simulink library "Lib_Piccolo"  (R2018b)
settings: Solver=VariableStepAuto  StartTime=0.0  StopTime=10.0  RelTol=1e-3
values from neighbouring files (symbols this model uses):
  AccelErrInt2Brakes = 0.15    [SimulationControlConfig16P.m]    (also in SimulationControlConfig16P_LEGACY.m; SimulationControlConfigTAILLESS.m = 0.2; SimulationControlConfigUTAIL.m = 0.2)
  AileronMax = 25    [SimulationControlConfig16P.m]    (also in SimulationControlConfig16P_LEGACY.m; SimulationControlConfigTAILLESS.m; SimulationControlConfigUTAIL.m)
  AileronPower = 0.00268    [SimulationControlConfig16P.m]    (also in SimulationControlConfig16P_LEGACY.m; SimulationControlConfigTAILLESS.m; SimulationControlConfigUTAIL.m)
  AileronSurfaceMax = 45    [SimulationControlConfig16P.m]    (also in SimulationControlConfig16P_LEGACY.m)
  AileronTrim = 0    [SimulationControlConfig16P.m]    (also in SimulationControlConfig16P_LEGACY.m; SimulationControlConfigTAILLESS.m; SimulationControlConfigUTAIL.m)
  Alt = 1000 + TerrainHeight    [SimulationStateConfig.m]
  AltCruise_m = testPlans(testIndx).terrainElevation * 0.3048 + 200    [SimulationControlConfig16P.m]    (also in SimulationControlConfigTAILLESS.m = 1083; SimulationControlConfigUTAIL.m = testPlans(testIndx).terrainElevation * 0.3048 + 152)
  AltitudeRate2PitchCmdIntegratorInit = 0.1    [SimulationControlPre.m]
  AltMax = 10000    [SimulationControlConfig16P.m]    (also in SimulationControlConfig16P_LEGACY.m; SimulationControlConfigTAILLESS.m; SimulationControlConfigUTAIL.m)
  AltMaxAccel = 1.25    [SimulationControlConfig16P.m]    (also in SimulationControlConfig16P_LEGACY.m = 0.9; SimulationControlConfigTAILLESS.m = 1.7; SimulationControlConfigUTAIL.m = 2)
  AltMin = 0    [SimulationControlConfig16P.m]    (also in SimulationControlConfig16P_LEGACY.m; SimulationControlConfigTAILLESS.m; SimulationControlConfigUTAIL.m)
  AltRateCmd2Pitch = 0.50    (= 0.5)    [SimulationControlConfig16P.m]    (also in SimulationControlConfig16P_LEGACY.m = 0.6; SimulationControlConfigTAILLESS.m = 0.2; SimulationControlConfigUTAIL.m = 0.3)
  AltRateError2Pitch = 0.40    (= 0.4)    [SimulationControlConfig16P.m]    (also in SimulationControlConfig16P_LEGACY.m; SimulationControlConfigTAILLESS.m = 0.55; SimulationControlConfigUTAIL.m = 0.55)
  AltRateErrorInt2Pitch = 0.50    (= 0.5)    [SimulationControlConfig16P.m]    (also in SimulationControlConfig16P_LEGACY.m = 0.45; SimulationControlConfigTAILLESS.m; SimulationControlConfigUTAIL.m = 0.75)
  AltRateLpfCutOff = 3    [SimulationControlConfig16P.m]    (also in SimulationControlConfig16P_LEGACY.m; SimulationControlConfigTAILLESS.m = 2; SimulationControlConfigUTAIL.m = 2)
  AutoNosegear2Rudder = 26    [SimulationControlConfig16P.m]    (also in SimulationControlConfig16P_LEGACY.m; SimulationControlConfigTAILLESS.m = 25.2; SimulationControlConfigUTAIL.m = 14)
  b = 5.54    [SimulationControlConfig16P.m]    (also in SimulationControlConfig16P_LEGACY.m; SimulationControlConfigTAILLESS.m = 2.37; SimulationControlConfigUTAIL.m = 2.37)
  Bank2AileronIntegratorInit = 0    [SimulationControlPre.m]
  BankMax_User = BankMax_User/180*pi    (= 0.523598775598)    [SimulationControlConfig16P.m]    (also in SimulationControlConfig16P_LEGACY.m; SimulationControlConfigTAILLESS.m = 0.610865238198; SimulationControlConfigUTAIL.m = 0.628318530718)
  baseLegFlaps = 20    [SimulationControlConfig16P.m]    (also in SimulationControlConfig16P_LEGACY.m = 0; SimulationControlConfigTAILLESS.m = 15; SimulationControlConfigUTAIL.m = 10)
  C = GeneticOpt.C    [SimulationCostFunction.m]
  c = Sw/b    (= 0.841696750903)    [SimulationControlConfig16P.m]    (also in SimulationControlConfig16P_LEGACY.m; SimulationControlConfigTAILLESS.m = 0.354008438819; SimulationControlConfigUTAIL.m = 0.354008438819)
  cell2WheelFactorMG = 5.98    [SimulationSensorConfig16P_LEGACY.m]
  cell2WheelFactorNG = 1    [SimulationSensorConfig16P_LEGACY.m]
  cellSatMaxMG = 15000    [SimulationSensorConfig16P.m]    (also in SimulationSensorConfig16P_LEGACY.m; SimulationSensorConfigTAILLESS7P.m; SimulationSensorConfigUTAIL7P.m)
  cellSatMaxNG = 1000    [SimulationSensorConfig16P.m]    (also in SimulationSensorConfig16P_LEGACY.m; SimulationSensorConfigTAILLESS7P.m; SimulationSensorConfigUTAIL7P.m)
  cellSatMinMG = -15000    [SimulationSensorConfig16P.m]    (also in SimulationSensorConfig16P_LEGACY.m; SimulationSensorConfigTAILLESS7P.m; SimulationSensorConfigUTAIL7P.m)
  cellSatMinNG = -1000    [SimulationSensorConfig16P.m]    (also in SimulationSensorConfig16P_LEGACY.m; SimulationSensorConfigTAILLESS7P.m; SimulationSensorConfigUTAIL7P.m)
  CL_Limit = CL_Max    (= 0.54)    [SimulationControlConfig16P.m]    (also in SimulationControlConfig16P_LEGACY.m; SimulationControlConfigTAILLESS.m; SimulationControlConfigUTAIL.m = 0.53)
  CL_Max = 0.54    [SimulationControlConfig16P.m]    (also in SimulationControlConfig16P_LEGACY.m; SimulationControlConfigTAILLESS.m; SimulationControlConfigUTAIL.m = 0.53)
  CL_Max_Nom = 0.465    [SimulationControlConfig16P.m]    (also in SimulationControlConfig16P_LEGACY.m; SimulationControlConfigTAILLESS.m = 0.39; SimulationControlConfigUTAIL.m)
  CL_Min = 0    [SimulationControlConfig16P.m]    (also in SimulationControlConfig16P_LEGACY.m; SimulationControlConfigTAILLESS.m; SimulationControlConfigUTAIL.m)
  ClimbMaxFraction = 0.35    [SimulationControlConfig16P.m]    (also in SimulationControlConfig16P_LEGACY.m = 0.24; SimulationControlConfigTAILLESS.m = 0.19; SimulationControlConfigUTAIL.m = 0.21)
  ClimboutMaxBank = 7.0    (= 7)    [SimulationControlConfig16P.m]    (also in SimulationControlConfig16P_LEGACY.m; SimulationControlConfigTAILLESS.m = 5; SimulationControlConfigUTAIL.m)
  ClimboutTimer = 7.0    (= 7)    [SimulationControlConfig16P.m]    (also in SimulationControlConfig16P_LEGACY.m; SimulationControlConfigTAILLESS.m; SimulationControlConfigUTAIL.m)
  dCl_per_dFlap = 0.005581818    [SimulationControlConfig16P.m]    (also in SimulationControlConfig16P_LEGACY.m = 0; SimulationControlConfigTAILLESS.m = 0; SimulationControlConfigUTAIL.m = 0)
  DecelerationCmd = 3.1    [SimulationControlConfig16P.m]    (also in SimulationControlConfig16P_LEGACY.m; SimulationControlConfigTAILLESS.m = 0.1; SimulationControlConfigUTAIL.m = 0.1)
  DeRotateLogicEndTimer = abs((NoseDownLimit_Deg-1)/DeRotateRamp_Dps)    [SimulationControlConfig16P.m]    (also in SimulationControlConfig16P_LEGACY.m; SimulationControlConfigTAILLESS.m; SimulationControlConfigUTAIL.m)
  DeRotateLogicHoldNoseUpTimer = 0.1    [SimulationControlConfig16P.m]    (also in SimulationControlConfig16P_LEGACY.m; SimulationControlConfigTAILLESS.m; SimulationControlConfigUTAIL.m)
  DeRotateLogicTimerTimeout = 2    [SimulationControlConfig16P.m]    (also in SimulationControlConfig16P_LEGACY.m; SimulationControlConfigTAILLESS.m; SimulationControlConfigUTAIL.m)
  DeRotateLowerCmdSaturation = 0    [SimulationControlConfig16P.m]    (also in SimulationControlConfig16P_LEGACY.m; SimulationControlConfigTAILLESS.m; SimulationControlConfigUTAIL.m)
  DeRotateRamp_Dps = 3    [SimulationControlConfig16P.m]    (also in SimulationControlConfig16P_LEGACY.m; SimulationControlConfigTAILLESS.m = 8; SimulationControlConfigUTAIL.m = 8)
  DeRotateUpperCmdSaturation = 7    [SimulationControlConfig16P.m]    (also in SimulationControlConfig16P_LEGACY.m; SimulationControlConfigTAILLESS.m; SimulationControlConfigUTAIL.m)
  DescentMaxFraction = 0.22    [SimulationControlConfig16P.m]    (also in SimulationControlConfig16P_LEGACY.m = 0.2; SimulationControlConfigTAILLESS.m = 0.17; SimulationControlConfigUTAIL.m = 0.17)
  DesktopSimTerrainOffset_m = 0.406    [SimulationAircraftConfig.m]
  downwindFlaps = 0    [SimulationControlConfig16P.m]    (also in SimulationControlConfig16P_LEGACY.m; SimulationControlConfigTAILLESS.m; SimulationControlConfigUTAIL.m)
  DP_init = 0.5*1.225*V_init^2    [SimulationControlConfig16P.m]    (also in SimulationControlConfig16P_LEGACY.m; SimulationControlConfigTAILLESS.m; SimulationControlConfigUTAIL.m)
  dscNoiseMG = 1    [SimulationSensorConfig16P_LEGACY.m]
  dscNoiseNG = 0.25    [SimulationSensorConfig16P_LEGACY.m]
  DSCnumBits = 24    [SimulationSensorConfig16P.m]    (also in SimulationSensorConfig16P_LEGACY.m; SimulationSensorConfigTAILLESS7P.m; SimulationSensorConfigUTAIL7P.m)
  DSCRangeMaxMG = 15000    [SimulationSensorConfig16P.m]    (also in SimulationSensorConfig16P_LEGACY.m; SimulationSensorConfigTAILLESS7P.m; SimulationSensorConfigUTAIL7P.m)
  DSCRangeMaxNG = 1000    [SimulationSensorConfig16P.m]    (also in SimulationSensorConfig16P_LEGACY.m; SimulationSensorConfigTAILLESS7P.m; SimulationSensorConfigUTAIL7P.m)
  DSCRangeMinMG = -15000    [SimulationSensorConfig16P.m]    (also in SimulationSensorConfig16P_LEGACY.m; SimulationSensorConfigTAILLESS7P.m; SimulationSensorConfigUTAIL7P.m)
  DSCRangeMinNG = -1000    [SimulationSensorConfig16P.m]    (also in SimulationSensorConfig16P_LEGACY.m; SimulationSensorConfigTAILLESS7P.m; SimulationSensorConfigUTAIL7P.m)
  dt = DLLSim.dt    [SimulationTimeStep.m]    (also in SimulationTrim.m = 0.02)
  EarlyTouchdownThreshold = 3.0    (= 3)    [SimulationControlConfig16P.m]    (also in SimulationControlConfig16P_LEGACY.m; SimulationControlConfigTAILLESS.m = 2.2; SimulationControlConfigUTAIL.m = 2.5)
  ElevatorDeflectionRate = 15    [SimulationControlConfig16P.m]    (also in SimulationControlConfig16P_LEGACY.m = 12; SimulationControlConfigTAILLESS.m = 10; SimulationControlConfigUTAIL.m = 12)
  ElevatorMax = 25    [SimulationControlConfig16P.m]    (also in SimulationControlConfig16P_LEGACY.m; SimulationControlConfigTAILLESS.m; SimulationControlConfigUTAIL.m)
  ElevatorPower = -0.002209    [SimulationControlConfig16P.m]    (also in SimulationControlConfig16P_LEGACY.m; SimulationControlConfigTAILLESS.m = -0.002956; SimulationControlConfigUTAIL.m = -0.00205983)
  ElevatorTrim = -3.5    [SimulationControlConfig16P.m]    (also in SimulationControlConfig16P_LEGACY.m; SimulationControlConfigTAILLESS.m = -6; SimulationControlConfigUTAIL.m = -8)
  elevonBias = 0    [SimulationControlConfig16P.m]    (also in SimulationControlConfig16P_LEGACY.m; SimulationControlConfigTAILLESS.m; SimulationControlConfigUTAIL.m)
  Enable_TAS_Protection = 0    [SimulationControlConfig16P.m]    (also in SimulationControlConfig16P_LEGACY.m; SimulationControlConfigTAILLESS.m; SimulationControlConfigUTAIL.m)
  EnableCrossTrackAbort = 1    [SimulationControlConfig16P.m]    (also in SimulationControlConfigTAILLESS.m; SimulationControlConfigUTAIL.m)
  EnergyBandwidth = 0.02    [SimulationControlConfig16P.m]    (also in SimulationControlConfig16P_LEGACY.m; SimulationControlConfigTAILLESS.m = 0.06; SimulationControlConfigUTAIL.m = 0.06)
  EngineLhFuelCut = 0    [SimulationAircraftConfig.m]
  EngineRhFuelCut = 0    [SimulationAircraftConfig.m]
  FastThrottleRate = 0.075    [SimulationControlConfig16P.m]    (also in SimulationControlConfig16P_LEGACY.m = 0.05; SimulationControlConfigTAILLESS.m = 0.1; SimulationControlConfigUTAIL.m = 0.1)
  FilterWarmUpTime = 2    [SimulationSensorConfig16P.m]    (also in SimulationSensorConfig16P_LEGACY.m; SimulationSensorConfigTAILLESS7P.m; SimulationSensorConfigUTAIL7P.m)
  finalApproachFlaps = 20    [SimulationControlConfig16P.m]    (also in SimulationControlConfig16P_LEGACY.m = 0; SimulationControlConfigTAILLESS.m = 22; SimulationControlConfigUTAIL.m = 10)
  FinalDescentSlope_Deg = testPlans(testIndx).descentSlope    [SimulationControlConfig16P.m]    (also in SimulationControlConfig16P_LEGACY.m; SimulationControlConfigTAILLESS.m; SimulationControlConfigUTAIL.m)
  flapMax = 0    [SimulationControlConfig16P.m]    (also in SimulationControlConfig16P_LEGACY.m; SimulationControlConfigTAILLESS.m; SimulationControlConfigUTAIL.m)
  flapRate = 7.5    [SimulationControlConfig16P.m]    (also in SimulationControlConfig16P_LEGACY.m; SimulationControlConfigTAILLESS.m = 6.6; SimulationControlConfigUTAIL.m)
  FlareHeight = 5    [SimulationControlConfig16P.m]    (also in SimulationControlConfig16P_LEGACY.m = 4.8; SimulationControlConfigTAILLESS.m = 2.5; SimulationControlConfigUTAIL.m = 2)
  FlareVerticalRate_mps = -0.4    [SimulationControlConfig16P.m]    (also in SimulationControlConfig16P_LEGACY.m = -0.5; SimulationControlConfigTAILLESS.m = -0.15; SimulationControlConfigUTAIL.m = -0.15)
  Fp_Aileron = 0.55*2*pi*RollRateLpfCutoff*dt    [SimulationControlConfig16P.m]    (also in SimulationControlConfig16P_LEGACY.m; SimulationControlConfigTAILLESS.m; SimulationControlConfigUTAIL.m)
  Fp_Alt = 0.55*AltBandwidth    (= 0.099)    [SimulationControlConfig16P.m]    (also in SimulationControlConfig16P_LEGACY.m; SimulationControlConfigTAILLESS.m = 0.587477826221; SimulationControlConfigUTAIL.m = 0.69115038379)
  Fp_AltRate = 0.55*2*pi*AltRateLpfCutOff*dt    [SimulationControlConfig16P.m]    (also in SimulationControlConfig16P_LEGACY.m; SimulationControlConfigTAILLESS.m; SimulationControlConfigUTAIL.m)
  Fp_Elevator = 0.55*2*pi*PitchRateLpfCutoff*dt    [SimulationControlConfig16P.m]    (also in SimulationControlConfig16P_LEGACY.m; SimulationControlConfigTAILLESS.m; SimulationControlConfigUTAIL.m)
  Fp_Energy = 0.55*2*pi*EnergyBandwidth    (= 0.069115038379)    [SimulationControlConfig16P.m]    (also in SimulationControlConfig16P_LEGACY.m; SimulationControlConfigTAILLESS.m = 0.207345115137; SimulationControlConfigUTAIL.m = 0.207345115137)
  Fp_Energy2 = 0.55*2*pi*EnergyBandwidth*dt    [SimulationControlConfig16P.m]    (also in SimulationControlConfig16P_LEGACY.m; SimulationControlConfigTAILLESS.m; SimulationControlConfigUTAIL.m)
  Fp_Pitch = 0.55*2*pi*PitchBandwidth    (= 2.76460153516)    [SimulationControlConfig16P.m]    (also in SimulationControlConfig16P_LEGACY.m = 3.11017672705; SimulationControlConfigTAILLESS.m = 3.80132711084; SimulationControlConfigUTAIL.m = 2.41902634326)
  Fp_Pitch_2 = 0.55*2*pi*PitchBandwidth*dt    [SimulationControlConfig16P.m]    (also in SimulationControlConfig16P_LEGACY.m; SimulationControlConfigTAILLESS.m; SimulationControlConfigUTAIL.m)
  Fp_Roll = RollBandwidth^2    (= 1)    [SimulationControlConfig16P.m]    (also in SimulationControlConfig16P_LEGACY.m = 1.44; SimulationControlConfigTAILLESS.m; SimulationControlConfigUTAIL.m)
  Fp_Rudder = 0.55*2*pi*YawRateLpfCutoff*dt    [SimulationControlConfig16P.m]    (also in SimulationControlConfig16P_LEGACY.m; SimulationControlConfigTAILLESS.m; SimulationControlConfigUTAIL.m)
  Fp_TAS = 0.55*2*pi*TASBandwidth    (= 0.103672557568)    [SimulationControlConfig16P.m]    (also in SimulationControlConfig16P_LEGACY.m; SimulationControlConfigTAILLESS.m = 0.172787595947; SimulationControlConfigUTAIL.m = 0.172787595947)
  Fp_TAS_Filter = 2*pi*TasLpfCutoff*dt    [SimulationControlConfig16P.m]    (also in SimulationControlConfig16P_LEGACY.m; SimulationControlConfigTAILLESS.m; SimulationControlConfigUTAIL.m)
  Fp_Turn = 0.55*2*pi*TurnErrLPFcutoff    (= 0.0345575191895)    [SimulationControlConfig16P.m]    (also in SimulationControlConfig16P_LEGACY.m; SimulationControlConfigTAILLESS.m = 0.172787595947; SimulationControlConfigUTAIL.m = 0.172787595947)
  Fp_TurnDerr = 0.55*2*pi*TurnDerivativeLPFcutoff    (= 0.0345575191895)    [SimulationControlConfig16P.m]    (also in SimulationControlConfig16P_LEGACY.m; SimulationControlConfigTAILLESS.m = 0.172787595947; SimulationControlConfigUTAIL.m = 0.172787595947)
  FTV = 3    [SimulationAircraftConfig.m]
  ftvStaticPositionError = 1/1.18    (= 0.847457627119)    [SimulationSensorConfig16P.m]    (also in SimulationSensorConfig16P_LEGACY.m; SimulationSensorConfigTAILLESS7P.m = 1; SimulationSensorConfigUTAIL7P.m = 1)
  g = 9.81    [SimulationStateConfig.m]
  GustSpd_Kts = testPlans(testIndx).gustSpd    [SimulationStateConfig.m]
  GustTriggerVal = testPlans(testIndx).gustTriggerVal    [SimulationStateConfig.m]
  HeadingErr2TurnRate = 0.5    [SimulationControlConfig16P.m]    (also in SimulationControlConfig16P_LEGACY.m; SimulationControlConfigTAILLESS.m; SimulationControlConfigUTAIL.m)
  HeadingErrDer2TurnRate = 0.3    [SimulationControlConfig16P.m]    (also in SimulationControlConfig16P_LEGACY.m; SimulationControlConfigTAILLESS.m; SimulationControlConfigUTAIL.m)
  IASbounce = IASstall*0.8    [SimulationControlPre.m]
  IAScruiseCMD = sqrt(2*m*9.81/(1.225*Sw*CL_cruise))    [SimulationControlConfig16P.m]    (also in SimulationControlConfig16P_LEGACY.m; SimulationControlConfigTAILLESS.m; SimulationControlConfigUTAIL.m)
  IASfinalCMD = 1.12 * IASmin    [SimulationControlConfig16P.m]    (also in SimulationControlConfig16P_LEGACY.m = 1.10 * IASmin; SimulationControlConfigTAILLESS.m = 1.10 * IASmin; SimulationControlConfigUTAIL.m = 1.15 * IASmin)
  IASflareCMD = IASstall    [SimulationControlConfig16P.m]    (also in SimulationControlConfig16P_LEGACY.m; SimulationControlConfigTAILLESS.m; SimulationControlConfigUTAIL.m)
  IASmax = 64    [SimulationControlConfig16P.m]    (also in SimulationControlConfig16P_LEGACY.m = 46; SimulationControlConfigTAILLESS.m = 38.58; SimulationControlConfigUTAIL.m = 35)
  IASmin = sqrt(2*m*9.81/(1.225*Sw*0.9*CL_Max_Nom))    [SimulationControlConfig16P.m]    (also in SimulationControlConfig16P_LEGACY.m; SimulationControlConfigTAILLESS.m; SimulationControlConfigUTAIL.m)
  IASshortCMD = IASstall    [SimulationControlConfig16P.m]    (also in SimulationControlConfig16P_LEGACY.m; SimulationControlConfigTAILLESS.m; SimulationControlConfigUTAIL.m)
  IASstall = sqrt(2*m*9.81/(1.225*Sw*CL_Max))    [SimulationControlConfig16P.m]    (also in SimulationControlConfig16P_LEGACY.m; SimulationControlConfigTAILLESS.m; SimulationControlConfigUTAIL.m)
  inFlight = 1    [SimulationControlConfig16P.m]    (also in SimulationControlConfigTAILLESS.m; SimulationControlConfigUTAIL.m)
  JetCatOffset = 5    [SimulationControlConfig16P.m]    (also in SimulationControlConfig16P_LEGACY.m)
  LaunchRollingElevator = -1.5    [SimulationControlConfig16P.m]    (also in SimulationControlConfig16P_LEGACY.m; SimulationControlConfigTAILLESS.m = 1; SimulationControlConfigUTAIL.m = 1)
  ldg_NosegearMax = 10    [SimulationControlConfig16P.m]    (also in SimulationControlConfig16P_LEGACY.m; SimulationControlConfigTAILLESS.m; SimulationControlConfigUTAIL.m)
  ldg_TrackVyErrInt2Nosegear = 0.1250    (= 0.125)    [SimulationControlConfig16P.m]    (also in SimulationControlConfig16P_LEGACY.m; SimulationControlConfigTAILLESS.m = 0.00714285714286; SimulationControlConfigUTAIL.m = 0.00714285714286)
  ldg_TrackVyErrPro2Nosegear = 0.35    [SimulationControlConfig16P.m]    (also in SimulationControlConfig16P_LEGACY.m; SimulationControlConfigTAILLESS.m = 0.0546666666667; SimulationControlConfigUTAIL.m = 0.0546666666667)
  ldg_TrackY2Vy = 0.07    [SimulationControlConfig16P.m]    (also in SimulationControlConfig16P_LEGACY.m; SimulationControlConfigTAILLESS.m = 0.17; SimulationControlConfigUTAIL.m = 0.17)
  ldg_Vy2NosegearScalingPower = 1.075    [SimulationControlConfig16P.m]    (also in SimulationControlConfig16P_LEGACY.m; SimulationControlConfigTAILLESS.m = 0.6; SimulationControlConfigUTAIL.m = 0.5)
  ldg_Y2VyScalingPower = 0.175    [SimulationControlConfig16P.m]    (also in SimulationControlConfig16P_LEGACY.m; SimulationControlConfigTAILLESS.m = 0; SimulationControlConfigUTAIL.m = 0)
  ldg_YawRate2Nosegear = 0.175    [SimulationControlConfig16P.m]    (also in SimulationControlConfig16P_LEGACY.m; SimulationControlConfigTAILLESS.m = 0.065; SimulationControlConfigUTAIL.m = 0.065)
  LiftSlope = 0.064285    [SimulationControlConfig16P.m]    (also in SimulationControlConfig16P_LEGACY.m; SimulationControlConfigTAILLESS.m = 0.058631; SimulationControlConfigUTAIL.m)
  LPFaileronInit = 0    [SimulationControlPre.m]
  LPFclestInit = 0    [SimulationControlPre.m]
  LPFenergyFFInit = 0    [SimulationControlPre.m]
  LPFtasInit = V_init + 2    [SimulationControlPre.m]
  LPFthrottleInit = ThrottleTrim    [SimulationControlPre.m]
  LPFturnErrInit = 0    [SimulationControlPre.m]
  ... (+115 more)
undefined symbols (not defined in the file or in its folder): abortFlag, alphaHPF, apmDelay, BRWNOUT, CRAWOR, CRAWUR, DiscIntNeverNeededParam, DLLSim, DLLSimStep, ECOMOR, ECOMUR, Fp_Tas, GustTrigger_HeightAgl_m, IPSTAT, LCINTEG, Ldg_Persist_Time, LOWER_FLAGS, MSG_ENABLE, NoiseStd, OLDVAL, OVERRIDE_ENABLE, OVERRIDE_VALUE, REBOOT, reversionEnable, revIASMax, revIASMin, revPitchMax, revPitchMin, revPitchRateMax, revRollMax, revRollRateMax, SAMPLE, SCALON, SensorModel, sigbuilder_block, Sim_Vx, Sim_Vy, Sim_Vz, Sim_Xpos, Sim_Ypos, Sim_Zpos, SYSOR, SYSUR, TARE, TEMPOR, TEMPUR, testIndx, testPlan, testPlans, Trim_piccoloInCmd, Trim_REFSI_FD_IN_nmodeCgShifterCmd_Ft, Trim_REFSI_FD_IN_nmodeFlapLhIBCmd_Deg, Trim_REFSI_FD_IN_nmodeFlapLhOBCmd_Deg, Trim_REFSI_FD_IN_nmodeFlapRhIBCmd_Deg, Trim_REFSI_FD_IN_nmodeFlapRhOBCmd_Deg, Trim_REFSI_FD_IN_nmodeSlatLhCmd_Deg, Trim_REFSI_FD_IN_nmodeSlatRhCmd_Deg, Trim_REFSI_FD_IN_nmodeSplrLhInbdCmd_Deg, Trim_REFSI_FD_IN_nmodeSplrLhOutbdCmd_Deg ... (+5)
libraries: simulink x866, aerolibconvert2 x60, $bdroot x52, aerolibatmos2 x5, dspswit3 x5, simulink_extras x4, dsparch4 x2, Lib_Piccolo_Alt x2, eeGeneralControl x1, dspindex x1
(part 27 of 44)

== system Lib_Piccolo/Ground Detection Systems/CL Detection Wrapper/CL Based Touchdown Detection Logic/Latch ==
  D : Inport
  Enable/!Rst : Inport  Port=2
  AND : Logic  IconShape=distinctive  AllPortsSameDT=off  OutDataTypeStr=boolean
  Constant : Constant
  OR : Logic  Operator=OR  IconShape=distinctive  AllPortsSameDT=off  OutDataTypeStr=boolean
  Switch : Switch  Criteria=u2 > Threshold  Threshold=0.5
  Unit Delay : UnitDelay  SampleTime=-1
  Q_Latched : Outport
  wires:
  Constant/1 -> Switch/1
  Enable/!Rst/1 -> AND/2
  AND/1 -> Switch/2
  OR/1 -> AND/1
  D/1 -> OR/1, Switch/3
  Switch/1 -> Unit Delay/1, Q_Latched/1
  Unit Delay/1 -> OR/2

== system Lib_Piccolo/Ground Detection Systems/CL Detection Wrapper/CL Based Touchdown Detection Logic/Latch1 ==
  D : Inport
  Enable/!Rst : Inport  Port=2
  AND : Logic  IconShape=distinctive  AllPortsSameDT=off  OutDataTypeStr=boolean
  Constant : Constant
  OR : Logic  Operator=OR  IconShape=distinctive  AllPortsSameDT=off  OutDataTypeStr=boolean
  Switch : Switch  Criteria=u2 > Threshold  Threshold=0.5
  Unit Delay : UnitDelay  SampleTime=-1
  Q_Latched : Outport
  wires:
  Constant/1 -> Switch/1
  Enable/!Rst/1 -> AND/2
  AND/1 -> Switch/2
  OR/1 -> AND/1
  D/1 -> OR/1, Switch/3
  Switch/1 -> Unit Delay/1, Q_Latched/1
  Unit Delay/1 -> OR/2

== system Lib_Piccolo/Ground Detection Systems/WoW Wrapper/Variant Subsystem/Load Cell WoW Model 1 ==
  note: These parameters are sent on the CMD and TELEM CAN Bus in the 328 ID Message
  note: Load Cell Model
  note: Ground Detection Logic
  note: DSC (Amplifier and ADC) Model
  note: CAN Bridge Data Acquisition and Processing
  note: Data Formatting for Piccolo Communications
  note: CANOpen transport delay from DSC to K2 is <1ms. A phase delay of 60-80ms for a given load measurement is occuring. Load phase Delay defined upstream at the input to this block.
  note: Relationship between measured load cell load and WoW load excluded since loads provided from FDM are already at wheel
  Piccolo_AP_Mode : Inport
  Bus Element In5 : Inport  Port=2  PortName=WoW_Bus_In  Element=ZgrndRhLbs
  Bus Element In4 : Inport  Port=2  PortName=WoW_Bus_In  Element=ZgrndLhLbs
  Bus Element In1 : Inport  Port=2  PortName=WoW_Bus_In  Element=ZgrndNgLbs
  ADC L : Quantizer  QuantizationInterval=(DSCRangeMaxMG-DSCRangeMinMG)/(2^DSCnumBits)
  ADC N : Quantizer  QuantizationInterval=(DSCRangeMaxNG-DSCRangeMinNG)/(2^DSCnumBits)
  ADC R : Quantizer  QuantizationInterval=(DSCRangeMaxMG-DSCRangeMinMG)/(2^DSCnumBits)
  Bus Creator : BusCreator  Inputs=2
  Bus Creator1 : BusCreator  Inputs=3
  Cell Saturation L : Saturate  UpperLimit=cellSatMaxMG/cell2WheelFactorMG  LowerLimit=cellSatMinMG/cell2WheelFactorMG
  Cell Saturation N : Saturate  UpperLimit=cellSatMaxNG/cell2WheelFactorNG  LowerLimit=cellSatMinNG/cell2WheelFactorNG
  Cell Saturation R : Saturate  UpperLimit=cellSatMaxMG/cell2WheelFactorMG  LowerLimit=cellSatMinMG/cell2WheelFactorMG
  Cell2WheelL : Gain
  Cell2WheelN : Gain
  Cell2WheelR : Gain
  Compare To Constant6 : simulink/Logic and Bit Operations/Compare To Constant  relop=>=  const=4  OutDataTypeStr=uint8
  DSC Noise L : RandomNumber  Variance=(dscNoiseMG/6)^2  Seed=20  SampleTime=dt
  DSC Noise N : RandomNumber  Variance=(dscNoiseNG/6)^2  Seed=20  SampleTime=dt
  DSC Noise R : RandomNumber  Variance=(dscNoiseMG/6)^2  Seed=10  SampleTime=dt
  DSC Saturation L : Saturate  UpperLimit=DSCRangeMaxMG/cell2WheelFactorMG  LowerLimit=DSCRangeMinMG/cell2WheelFactorMG
  DSC Saturation N : Saturate  UpperLimit=DSCRangeMaxNG/cell2WheelFactorNG  LowerLimit=DSCRangeMinNG/cell2WheelFactorNG
  DSC Saturation R : Saturate  UpperLimit=DSCRangeMaxMG/cell2WheelFactorMG  LowerLimit=DSCRangeMinMG/cell2WheelFactorMG
  Data Type Conversion : DataTypeConversion
  Data Type Conversion1 : DataTypeConversion
  Delay1 : Delay  DelayLength=WOWtransportDelay
  Delay2 : Delay  DelayLength=WOWtransportDelay
  Delay3 : Delay  DelayLength=WOWtransportDelay
  Force Conversion L : aerolibconvert2/Force Conversion  IU=lbf  OU=N
      settings: SourceProductName=Aerospace Blockset  SourceProductBaseCode=AE
  Force Conversion N : aerolibconvert2/Force Conversion  IU=lbf  OU=N
      settings: SourceProductName=Aerospace Blockset  SourceProductBaseCode=AE
  Force Conversion R : aerolibconvert2/Force Conversion  IU=lbf  OU=N
      settings: SourceProductName=Aerospace Blockset  SourceProductBaseCode=AE
  Gain : Gain  Gain=100
  Ground : Ground
  LPF L : Subsystem  mask{Cutoff=SensorModel.WOW.Cell.fc, Init=0}
      mask prompts: Cutoff "Cutoff Frequency [Hz]"; Init "Initial Condition"
  LPF N : Subsystem  mask{Cutoff=SensorModel.WOW.Cell.fc, Init=0}
      mask prompts: Cutoff "Cutoff Frequency [Hz]"; Init "Initial Condition"
  LPF R : Subsystem  mask{Cutoff=SensorModel.WOW.Cell.fc, Init=0}
      mask prompts: Cutoff "Cutoff Frequency [Hz]"; Init "Initial Condition"
  Landing Configuration : Subsystem
  Re-Encoding L : Quantizer  QuantizationInterval=(satMaxMG-satMinMG)/(2^numBits)
  Re-Encoding N : Quantizer  QuantizationInterval=(satMaxNG-satMinNG)/(2^numBits)
  Re-Encoding R : Quantizer  QuantizationInterval=(satMaxMG-satMinMG)/(2^numBits)
  Signal Specification1 : SignalSpecification  Dimensions=[1 1]  SampleTime=dt
  Signal Specification2 : SignalSpecification  Dimensions=[1 1]  SampleTime=dt
  Signal Specification3 : SignalSpecification  Dimensions=[1 1]  SampleTime=dt
  Software Saturation L : Saturate  UpperLimit=satMaxMG  LowerLimit=satMinMG
  Software Saturation N : Saturate  UpperLimit=satMaxMG  LowerLimit=satMinMG
  Software Saturation R : Saturate  UpperLimit=satMaxMG  LowerLimit=satMinMG
  Sum : Sum  Inputs=|++
  Sum1 : Sum  Inputs=|++
  Sum2 : Sum  Inputs=|++
  Switch : Switch  Criteria=u2 > Threshold
  T/O Configuration : Subsystem
  WOW_Bus_Out : Outport
  tag scope: Sim_WOW_L_N=global, Sim_WOW_NG_N=global, Sim_WOW_R_N=global
  wires:
  Cell2WheelN/1 -> LPF N/1(Input)  "Sim.WOW_NG_N"
  Re-Encoding N/1 -> Cell2WheelN/1
  Software Saturation N/1 -> Re-Encoding N/1
  Signal Specification3/1 -> Software Saturation N/1
  Delay3/1 -> Signal Specification3/1
  Force Conversion R/1 -> Cell Saturation R/1
  Force Conversion L/1 -> Cell Saturation L/1
  Force Conversion N/1 -> Cell Saturation N/1
  ADC N/1 -> Delay3/1
  Cell Saturation N/1 -> DSC Saturation N/1
  DSC Noise N/1 -> Sum2/2
  Sum2/1 -> ADC N/1
  DSC Saturation N/1 -> Sum2/1
  Bus Element In1/1 -> Force Conversion N/1
  Cell2WheelR/1 -> LPF R/1(Input)  "Sim.WOW_R_N"
  Cell2WheelL/1 -> LPF L/1(Input)  "Sim.WOW_L_N"
  DSC Noise L/1 -> Sum/2
  Sum/1 -> ADC L/1
  DSC Saturation L/1 -> Sum/1
  DSC Noise R/1 -> Sum1/2
  DSC Saturation R/1 -> Sum1/1
  Sum1/1 -> ADC R/1
  Delay2/1 -> Signal Specification2/1
  ADC R/1 -> Delay2/1
  Delay1/1 -> Signal Specification1/1
  ADC L/1 -> Delay1/1
  Re-Encoding R/1 -> Cell2WheelR/1
  Re-Encoding L/1 -> Cell2WheelL/1
  Software Saturation R/1 -> Re-Encoding R/1
  Signal Specification2/1 -> Software Saturation R/1
  Software Saturation L/1 -> Re-Encoding L/1
  Signal Specification1/1 -> Software Saturation L/1
  Cell Saturation R/1 -> DSC Saturation R/1
  Cell Saturation L/1 -> DSC Saturation L/1
  Data Type Conversion1/1 -> Bus Creator/2  "WoWPcnt"
  Gain/1 -> Data Type Conversion1/1
  Data Type Conversion/1 -> Bus Creator/1  "ContactBool"
  Bus Creator/1 -> WOW_Bus_Out/1
  Bus Element In5/1 -> Force Conversion R/1
  Bus Element In4/1 -> Force Conversion L/1
  LPF R/1(Output) -> [Sim_WOW_R_N], Bus Creator1/3  "Sim.WOW_Filt_R"
  LPF L/1(Output) -> Bus Creator1/2, [Sim_WOW_L_N]  "Sim.WOW_Filt_L"
  LPF N/1(Output) -> Bus Creator1/1, [Sim_WOW_NG_N]  "Sim.WOW_Filt_NG"
  Bus Creator1/1 -> T/O Configuration/1(Sim.WOW_Filt), Landing Configuration/1(Sim.WOW_Filt)
  Landing Configuration/1(ContactBool) -> Switch/1
  Switch/1 -> Data Type Conversion/1, Gain/1
  T/O Configuration/1(ContactBool) -> Switch/3
  Piccolo_AP_Mode/1 -> Compare To Constant6/1
  Compare To Constant6/1 -> Switch/2
  Ground/1 -> LPF R/2(Reset), LPF N/2(Reset), LPF L/2(Reset)

== system Lib_Piccolo/Ground Detection Systems/WoW Wrapper/Variant Subsystem/Load Cell WoW Model 1 16P5 AsFlown 2022 ==
  note: Relationship between measured load cell load and WoW load excluded since loads provided from FDM are already at wheel
  note: CANOpen transport delay from DSC to K2 is <1ms. A phase delay of 60-80ms for a given load measurement is occuring. Load phase Delay defined upstream at the input to this block.
  note: Data Formatting for Piccolo Communications
  note: CAN Bridge Data Acquisition and Processing
  note: DSC (Amplifier and ADC) Model
  note: Ground Detection Logic
  note: Load Cell Model
  note: These parameters are sent on the CMD and TELEM CAN Bus in the 328 ID Message
  Piccolo_AP_Mode : Inport
  Bus Element In5 : Inport  Port=2  PortName=WoW_Bus_In  Element=ZgrndRhLbs
  Bus Element In4 : Inport  Port=2  PortName=WoW_Bus_In  Element=ZgrndLhLbs
  Bus Element In1 : Inport  Port=2  PortName=WoW_Bus_In  Element=ZgrndNgLbs
  ADC L : Quantizer  QuantizationInterval=(DSCRangeMaxMG-DSCRangeMinMG)/(2^DSCnumBits)
  ADC N : Quantizer  QuantizationInterval=(DSCRangeMaxNG-DSCRangeMinNG)/(2^DSCnumBits)
  ADC R : Quantizer  QuantizationInterval=(DSCRangeMaxMG-DSCRangeMinMG)/(2^DSCnumBits)
  Bus Creator : BusCreator  Inputs=2
  Bus Creator1 : BusCreator  Inputs=3
  Cell Saturation L : Saturate  UpperLimit=cellSatMaxMG/cell2WheelFactorMG  LowerLimit=cellSatMinMG/cell2WheelFactorMG
  Cell Saturation N : Saturate  UpperLimit=cellSatMaxNG/cell2WheelFactorNG  LowerLimit=cellSatMinNG/cell2WheelFactorNG
  Cell Saturation R : Saturate  UpperLimit=cellSatMaxMG/cell2WheelFactorMG  LowerLimit=cellSatMinMG/cell2WheelFactorMG
  Cell2WheelL : Gain
  Cell2WheelN : Gain
  Cell2WheelR : Gain
  Compare To Constant6 : simulink/Logic and Bit Operations/Compare To Constant  relop=>=  const=4  OutDataTypeStr=uint8
  DSC Noise L : RandomNumber  Variance=(dscNoiseMG/6)^2  Seed=20  SampleTime=dt
  DSC Noise N : RandomNumber  Variance=(dscNoiseNG/6)^2  Seed=20  SampleTime=dt
  DSC Noise R : RandomNumber  Variance=(dscNoiseMG/6)^2  Seed=10  SampleTime=dt
  DSC Saturation L : Saturate  UpperLimit=DSCRangeMaxMG/cell2WheelFactorMG  LowerLimit=DSCRangeMinMG/cell2WheelFactorMG
  DSC Saturation N : Saturate  UpperLimit=DSCRangeMaxNG/cell2WheelFactorNG  LowerLimit=DSCRangeMinNG/cell2WheelFactorNG
  DSC Saturation R : Saturate  UpperLimit=DSCRangeMaxMG/cell2WheelFactorMG  LowerLimit=DSCRangeMinMG/cell2WheelFactorMG
  Data Type Conversion : DataTypeConversion
  Data Type Conversion1 : DataTypeConversion
  Delay1 : Delay
  Delay2 : Delay
  Delay3 : Delay
  Force Conversion L : aerolibconvert2/Force Conversion  IU=lbf  OU=N
      settings: SourceProductName=Aerospace Blockset  SourceProductBaseCode=AE
  Force Conversion N : aerolibconvert2/Force Conversion  IU=lbf  OU=N
      settings: SourceProductName=Aerospace Blockset  SourceProductBaseCode=AE
  Force Conversion R : aerolibconvert2/Force Conversion  IU=lbf  OU=N
      settings: SourceProductName=Aerospace Blockset  SourceProductBaseCode=AE
  Gain : Gain  Gain=100
  Ground : Ground
  LPF L : Subsystem  mask{Cutoff=2, Init=0}
      mask prompts: Cutoff "Cutoff Frequency [Hz]"; Init "Initial Condition"
  LPF N : Subsystem  mask{Cutoff=2, Init=0}
      mask prompts: Cutoff "Cutoff Frequency [Hz]"; Init "Initial Condition"
  LPF R : Subsystem  mask{Cutoff=2, Init=0}
      mask prompts: Cutoff "Cutoff Frequency [Hz]"; Init "Initial Condition"
  Landing Configuration : Subsystem
  Re-Encoding L : Quantizer  QuantizationInterval=(satMaxMG-satMinMG)/(2^numBits)
  Re-Encoding N : Quantizer  QuantizationInterval=(satMaxNG-satMinNG)/(2^numBits)
  Re-Encoding R : Quantizer  QuantizationInterval=(satMaxMG-satMinMG)/(2^numBits)
  Signal Specification1 : SignalSpecification  Dimensions=[1 1]  SampleTime=dt
  Signal Specification2 : SignalSpecification  Dimensions=[1 1]  SampleTime=dt
  Signal Specification3 : SignalSpecification  Dimensions=[1 1]  SampleTime=dt
  Software Saturation L : Saturate  UpperLimit=satMaxMG  LowerLimit=satMinMG
  Software Saturation N : Saturate  UpperLimit=satMaxMG  LowerLimit=satMinMG
  Software Saturation R : Saturate  UpperLimit=satMaxMG  LowerLimit=satMinMG
  Sum : Sum  Inputs=|++
  Sum1 : Sum  Inputs=|++
  Sum2 : Sum  Inputs=|++
  Switch : Switch  Criteria=u2 > Threshold
  T/O Configuration : Subsystem
  WOW_Bus_Out : Outport
  tag scope: Sim_WOW_L_N=global, Sim_WOW_NG_N=global, Sim_WOW_R_N=global
  wires:
  Ground/1 -> LPF L/2(Reset), LPF N/2(Reset), LPF R/2(Reset)
  Compare To Constant6/1 -> Switch/2
  Piccolo_AP_Mode/1 -> Compare To Constant6/1
  T/O Configuration/1(ContactBool) -> Switch/3
  Switch/1 -> Gain/1, Data Type Conversion/1
  Landing Configuration/1(ContactBool) -> Switch/1
  Bus Creator1/1 -> Landing Configuration/1(Sim.WOW_Filt), T/O Configuration/1(Sim.WOW_Filt)
  LPF N/1(Output) -> [Sim_WOW_NG_N], Bus Creator1/1  "Sim.WOW_Filt_NG"
  LPF L/1(Output) -> [Sim_WOW_L_N], Bus Creator1/2  "Sim.WOW_Filt_L"
  LPF R/1(Output) -> Bus Creator1/3, [Sim_WOW_R_N]  "Sim.WOW_Filt_R"
  Bus Element In4/1 -> Force Conversion L/1
  Bus Element In5/1 -> Force Conversion R/1
  Bus Creator/1 -> WOW_Bus_Out/1
  Data Type Conversion/1 -> Bus Creator/1  "ContactBool"
  Gain/1 -> Data Type Conversion1/1
  Data Type Conversion1/1 -> Bus Creator/2  "WoWPcnt"
  Cell Saturation L/1 -> DSC Saturation L/1
  Cell Saturation R/1 -> DSC Saturation R/1
  Signal Specification1/1 -> Software Saturation L/1
  Software Saturation L/1 -> Re-Encoding L/1
  Signal Specification2/1 -> Software Saturation R/1
  Software Saturation R/1 -> Re-Encoding R/1
  Re-Encoding L/1 -> Cell2WheelL/1
  Re-Encoding R/1 -> Cell2WheelR/1
  ADC L/1 -> Delay1/1
  Delay1/1 -> Signal Specification1/1
  ADC R/1 -> Delay2/1
  Delay2/1 -> Signal Specification2/1
  Sum1/1 -> ADC R/1
  DSC Saturation R/1 -> Sum1/1
  DSC Noise R/1 -> Sum1/2
  DSC Saturation L/1 -> Sum/1
  Sum/1 -> ADC L/1
  DSC Noise L/1 -> Sum/2
  Cell2WheelL/1 -> LPF L/1(Input)  "Sim.WOW_L_N"
  Cell2WheelR/1 -> LPF R/1(Input)  "Sim.WOW_R_N"
  Bus Element In1/1 -> Force Conversion N/1
  DSC Saturation N/1 -> Sum2/1
  Sum2/1 -> ADC N/1
  DSC Noise N/1 -> Sum2/2
  Cell Saturation N/1 -> DSC Saturation N/1
  ADC N/1 -> Delay3/1
  Force Conversion N/1 -> Cell Saturation N/1
  Force Conversion L/1 -> Cell Saturation L/1
  Force Conversion R/1 -> Cell Saturation R/1
  Delay3/1 -> Signal Specification3/1
  Signal Specification3/1 -> Software Saturation N/1
  Software Saturation N/1 -> Re-Encoding N/1
  Re-Encoding N/1 -> Cell2WheelN/1
  Cell2WheelN/1 -> LPF N/1(Input)  "Sim.WOW_NG_N"

== system Lib_Piccolo/Ground Detection Systems/WoW Wrapper/Variant Subsystem/Load Cell WoW Model 1 7P AsFlown ==
  note: These parameters are sent on the CMD and TELEM CAN Bus in the 328 ID Message
  note: Load Cell Model
  note: Ground Detection Logic
  note: DSC (Amplifier and ADC) Model
  note: CAN Bridge Data Acquisition and Processing
  note: Data Formatting for Piccolo Communications
  note: CANOpen transport delay from DSC to K2 is <1ms. A phase delay of 60-80ms for a given load measurement is occuring. Load phase Delay defined upstream at the input to this block.
  note: Relationship between measured load cell load and WoW load excluded since loads provided from FDM are already at wheel
  Piccolo_AP_Mode : Inport
  Bus Element In5 : Inport  Port=2  PortName=WoW_Bus_In  Element=ZgrndRhLbs
  Bus Element In4 : Inport  Port=2  PortName=WoW_Bus_In  Element=ZgrndLhLbs
  Bus Element In1 : Inport  Port=2  PortName=WoW_Bus_In  Element=ZgrndNgLbs
  ADC L : Quantizer  QuantizationInterval=(DSCRangeMaxMG-DSCRangeMinMG)/(2^DSCnumBits)
  ADC N : Quantizer  QuantizationInterval=(DSCRangeMaxNG-DSCRangeMinNG)/(2^DSCnumBits)
  ADC R : Quantizer  QuantizationInterval=(DSCRangeMaxMG-DSCRangeMinMG)/(2^DSCnumBits)
  Bus Creator : BusCreator  Inputs=2
  Bus Creator1 : BusCreator  Inputs=3
  Cell Saturation L : Saturate  UpperLimit=cellSatMaxMG/cell2WheelFactorMG  LowerLimit=cellSatMinMG/cell2WheelFactorMG
  Cell Saturation N : Saturate  UpperLimit=cellSatMaxNG/cell2WheelFactorNG  LowerLimit=cellSatMinNG/cell2WheelFactorNG
  Cell Saturation R : Saturate  UpperLimit=cellSatMaxMG/cell2WheelFactorMG  LowerLimit=cellSatMinMG/cell2WheelFactorMG
  Cell2WheelL : Gain
  Cell2WheelN : Gain
  Cell2WheelR : Gain
  Compare To Constant6 : simulink/Logic and Bit Operations/Compare To Constant  relop=>=  const=4  OutDataTypeStr=uint8
  DSC Noise L : RandomNumber  Variance=(dscNoiseMG/6)^2  Seed=20  SampleTime=dt
  DSC Noise N : RandomNumber  Variance=(dscNoiseNG/6)^2  Seed=20  SampleTime=dt
  DSC Noise R : RandomNumber  Variance=(dscNoiseMG/6)^2  Seed=10  SampleTime=dt
  DSC Saturation L : Saturate  UpperLimit=DSCRangeMaxMG/cell2WheelFactorMG  LowerLimit=DSCRangeMinMG/cell2WheelFactorMG
  DSC Saturation N : Saturate  UpperLimit=DSCRangeMaxNG/cell2WheelFactorNG  LowerLimit=DSCRangeMinNG/cell2WheelFactorNG
  DSC Saturation R : Saturate  UpperLimit=DSCRangeMaxMG/cell2WheelFactorMG  LowerLimit=DSCRangeMinMG/cell2WheelFactorMG
  Data Type Conversion : DataTypeConversion
  Data Type Conversion1 : DataTypeConversion
  Delay1 : Delay
  Delay2 : Delay
  Delay3 : Delay
  Force Conversion L : aerolibconvert2/Force Conversion  IU=lbf  OU=N
      settings: SourceProductName=Aerospace Blockset  SourceProductBaseCode=AE
  Force Conversion N : aerolibconvert2/Force Conversion  IU=lbf  OU=N
      settings: SourceProductName=Aerospace Blockset  SourceProductBaseCode=AE
  Force Conversion R : aerolibconvert2/Force Conversion  IU=lbf  OU=N
      settings: SourceProductName=Aerospace Blockset  SourceProductBaseCode=AE
  Gain : Gain  Gain=100
  Ground : Ground
  LPF L : Subsystem  mask{Cutoff=2, Init=0}
      mask prompts: Cutoff "Cutoff Frequency [Hz]"; Init "Initial Condition"
  LPF N : Subsystem  mask{Cutoff=2, Init=0}
      mask prompts: Cutoff "Cutoff Frequency [Hz]"; Init "Initial Condition"
  LPF R : Subsystem  mask{Cutoff=2, Init=0}
      mask prompts: Cutoff "Cutoff Frequency [Hz]"; Init "Initial Condition"
  Landing Configuration : Subsystem
  Re-Encoding L : Quantizer  QuantizationInterval=(satMaxMG-satMinMG)/(2^numBits)
  Re-Encoding N : Quantizer  QuantizationInterval=(satMaxNG-satMinNG)/(2^numBits)
  Re-Encoding R : Quantizer  QuantizationInterval=(satMaxMG-satMinMG)/(2^numBits)
  Signal Specification1 : SignalSpecification  Dimensions=[1 1]  SampleTime=dt
  Signal Specification2 : SignalSpecification  Dimensions=[1 1]  SampleTime=dt
  Signal Specification3 : SignalSpecification  Dimensions=[1 1]  SampleTime=dt
  Software Saturation L : Saturate  UpperLimit=satMaxMG  LowerLimit=satMinMG
  Software Saturation N : Saturate  UpperLimit=satMaxMG  LowerLimit=satMinMG
  Software Saturation R : Saturate  UpperLimit=satMaxMG  LowerLimit=satMinMG
  Sum : Sum  Inputs=|++
  Sum1 : Sum  Inputs=|++
  Sum2 : Sum  Inputs=|++
  Switch : Switch  Criteria=u2 > Threshold
  T/O Configuration : Subsystem
  WOW_Bus_Out : Outport
  tag scope: Sim_WOW_L_N=global, Sim_WOW_NG_N=global, Sim_WOW_R_N=global
  wires:
  Cell2WheelN/1 -> LPF N/1(Input)  "Sim.WOW_NG_N"
  Re-Encoding N/1 -> Cell2WheelN/1
  Software Saturation N/1 -> Re-Encoding N/1
  Signal Specification3/1 -> Software Saturation N/1
  Delay3/1 -> Signal Specification3/1
  Force Conversion R/1 -> Cell Saturation R/1
  Force Conversion L/1 -> Cell Saturation L/1
  Force Conversion N/1 -> Cell Saturation N/1
  ADC N/1 -> Delay3/1
  Cell Saturation N/1 -> DSC Saturation N/1
  DSC Noise N/1 -> Sum2/2
  Sum2/1 -> ADC N/1
  DSC Saturation N/1 -> Sum2/1
  Bus Element In1/1 -> Force Conversion N/1
  Cell2WheelR/1 -> LPF R/1(Input)  "Sim.WOW_R_N"
  Cell2WheelL/1 -> LPF L/1(Input)  "Sim.WOW_L_N"
  DSC Noise L/1 -> Sum/2
  Sum/1 -> ADC L/1
  DSC Saturation L/1 -> Sum/1
  DSC Noise R/1 -> Sum1/2
  DSC Saturation R/1 -> Sum1/1
  Sum1/1 -> ADC R/1
  Delay2/1 -> Signal Specification2/1
  ADC R/1 -> Delay2/1
  Delay1/1 -> Signal Specification1/1
  ADC L/1 -> Delay1/1
  Re-Encoding R/1 -> Cell2WheelR/1
  Re-Encoding L/1 -> Cell2WheelL/1
  Software Saturation R/1 -> Re-Encoding R/1
  Signal Specification2/1 -> Software Saturation R/1
  Software Saturation L/1 -> Re-Encoding L/1
  Signal Specification1/1 -> Software Saturation L/1
  Cell Saturation R/1 -> DSC Saturation R/1
  Cell Saturation L/1 -> DSC Saturation L/1
  Data Type Conversion1/1 -> Bus Creator/2  "WoWPcnt"
  Gain/1 -> Data Type Conversion1/1
  Data Type Conversion/1 -> Bus Creator/1  "ContactBool"
  Bus Creator/1 -> WOW_Bus_Out/1
  Bus Element In5/1 -> Force Conversion R/1
  Bus Element In4/1 -> Force Conversion L/1
  LPF R/1(Output) -> [Sim_WOW_R_N], Bus Creator1/3  "Sim.WOW_Filt_R"
  LPF L/1(Output) -> Bus Creator1/2, [Sim_WOW_L_N]  "Sim.WOW_Filt_L"
  LPF N/1(Output) -> Bus Creator1/1, [Sim_WOW_NG_N]  "Sim.WOW_Filt_NG"
  Bus Creator1/1 -> T/O Configuration/1(Sim.WOW_Filt), Landing Configuration/1(Sim.WOW_Filt)
  Landing Configuration/1(ContactBool) -> Switch/1
  Switch/1 -> Data Type Conversion/1, Gain/1
  T/O Configuration/1(ContactBool) -> Switch/3
  Piccolo_AP_Mode/1 -> Compare To Constant6/1
  Compare To Constant6/1 -> Switch/2
  Ground/1 -> LPF R/2(Reset), LPF N/2(Reset), LPF L/2(Reset)

== system Lib_Piccolo/Ground Detection Systems/WoW Wrapper/Variant Subsystem/Load Cell WoW Model 16 ==
  note: Data Formatting for Piccolo Communications
  note: DSC Model
  note: Inputs to WOW block are 32-bit float (IEEE 754) direct from DSC with appropriate cell scaling applied. Re-encoded integer loads are only used for telemetry output.
  note: CANOpen transport delay from DSC to K2 is <1ms. Addtional delay here also accounts for worst case asynchronicity between DSC PDO and K2 sampling. Load phase delay defined in workspace.
  note: These signals are sent on the CMD and TELEM CAN Bus in the 0x3280000 ID Message
  note: Scaling relationship between measured load cell load and WoW load excluded since loads provided from FDM are already at wheel
  note: K2 Data Acquisition and Processing
  note: Load Cell Model
  Piccolo_AP_Mode : Inport
  Bus Element In5 : Inport  Port=2  PortName=WoW_Bus_In  Element=ZgrndRhLbs
  Bus Element In4 : Inport  Port=2  PortName=WoW_Bus_In  Element=ZgrndLhLbs
  Bus Element In1 : Inport  Port=2  PortName=WoW_Bus_In  Element=ZgrndNgLbs
  Bus Creator : BusCreator  Inputs=2
  Bus Creator1 : BusCreator  Inputs=3
  Cell to Wheel Load MGL : Gain
  Cell to Wheel Load MGR : Gain
  Cell to Wheel Load NG : Gain
  Conversion - MGL : $bdroot/Ground Detection Systems/WoW Wrapper/Variant Subsystem/Load Cell WoW Model 18/Conversion - NG  SystemSampleTime=-1  Latency=0  AutoFrameSizeCalculation=off
  Conversion - MGR : $bdroot/Ground Detection Systems/WoW Wrapper/Variant Subsystem/Load Cell WoW Model 18/Conversion - NG  SystemSampleTime=-1  Latency=0  AutoFrameSizeCalculation=off
  Conversion - NG : $bdroot/Ground Detection Systems/WoW Wrapper/Variant Subsystem/Load Cell WoW Model 18/Conversion - NG  SystemSampleTime=-1  Latency=0  AutoFrameSizeCalculation=off
  DSC Noise L : RandomNumber  Variance=(SensorModel.WOW.Cell.dscNoiseMG/6)^2  Seed=20  SampleTime=dt
  DSC Noise N : RandomNumber  Variance=(SensorModel.WOW.Cell.dscNoiseNG/6)^2  Seed=10  SampleTime=dt
  DSC Noise R : RandomNumber  Variance=(SensorModel.WOW.Cell.dscNoiseMG/6)^2  Seed=30  SampleTime=dt
  Data Type Conversion : DataTypeConversion
  Data Type Conversion1 : DataTypeConversion
  Data Type L : DataTypeConversion  OutDataTypeStr=single
  Data Type N : DataTypeConversion  OutDataTypeStr=single
  Data Type R : DataTypeConversion  OutDataTypeStr=single
  Delay1 : Delay  DelayLength=SensorModel.WOW.Cell.WOWtransportDelay
  Delay2 : Delay  DelayLength=SensorModel.WOW.Cell.WOWtransportDelay
  Delay3 : Delay  DelayLength=SensorModel.WOW.Cell.WOWtransportDelay
  Gain : Gain  Gain=100
  Ground : Ground
  Quantization L : Quantizer  QuantizationInterval=(SensorModel.WOW.Cell.calibrationSlopeMG * (SensorModel.WOW.Cell.fullScaleRange/SensorModel.WOW.Cell.effectiveCounts)) / SensorModel.WOW.Cell.cell2WheelFactorMG
  Quantization N : Quantizer  QuantizationInterval=(SensorModel.WOW.Cell.calibrationSlopeNG * (SensorModel.WOW.Cell.fullScaleRange/SensorModel.WOW.Cell.effectiveCounts)) / SensorModel.WOW.Cell.cell2WheelFactorNG
  Quantization R : Quantizer  QuantizationInterval=(SensorModel.WOW.Cell.calibrationSlopeMG * (SensorModel.WOW.Cell.fullScaleRange/SensorModel.WOW.Cell.effectiveCounts)) / SensorModel.WOW.Cell.cell2WheelFactorMG
  Re-Encoding L : Quantizer  QuantizationInterval=(SensorModel.WOW.Cell.satMaxMG-SensorModel.WOW.Cell.satMinMG)/(2^SensorModel.WOW.Cell.numBits)
  Re-Encoding N : Quantizer  QuantizationInterval=(SensorModel.WOW.Cell.satMaxNG-SensorModel.WOW.Cell.satMinNG)/(2^SensorModel.WOW.Cell.numBits)
  Re-Encoding R : Quantizer  QuantizationInterval=(SensorModel.WOW.Cell.satMaxMG-SensorModel.WOW.Cell.satMinMG)/(2^SensorModel.WOW.Cell.numBits)  LinearizeAsGain=off
  Signal Specification L : SignalSpecification  OutDataTypeStr=single  Dimensions=[1 1]  SampleTime=dt
  Signal Specification N : SignalSpecification  OutDataTypeStr=single  Dimensions=[1 1]  SampleTime=dt
  Signal Specification R : SignalSpecification  OutDataTypeStr=single  Dimensions=[1 1]  SampleTime=dt
  Software Saturation L : Saturate  UpperLimit=SensorModel.WOW.Cell.satMaxMG  LowerLimit=SensorModel.WOW.Cell.satMinMG
  Software Saturation N : Saturate  UpperLimit=SensorModel.WOW.Cell.satMaxNG  LowerLimit=SensorModel.WOW.Cell.satMinNG
  Software Saturation R : Saturate  UpperLimit=SensorModel.WOW.Cell.satMaxMG  LowerLimit=SensorModel.WOW.Cell.satMinMG
  Subsystem : Subsystem
  Sum : Sum  Inputs=|++
  Sum1 : Sum  Inputs=|++
  Sum2 : Sum  Inputs=|++
  Terminator : Terminator
  Wheel to Cell Load MGL : Gain  Gain=SensorModel.WOW.Cell.cell2WheelFactorMG
  Wheel to Cell Load MGR : Gain  Gain=SensorModel.WOW.Cell.cell2WheelFactorMG
  Wheel to Cell Load NG : Gain  Gain=SensorModel.WOW.Cell.cell2WheelFactorNG
  WOW_Bus_Out : Outport
  tag scope: Sim_WOW_L_N=global, Sim_WOW_NG_N=global, Sim_WOW_R_N=global
  wires:
  Subsystem/4(Sim.WOW_Filt_R) -> [Sim_WOW_R_N]
  Subsystem/2(Sim.WOW_Filt_L) -> [Sim_WOW_L_N]
  Subsystem/1(Sim.WOW_Filt_NG) -> [Sim_WOW_NG_N]
  Piccolo_AP_Mode/1 -> Subsystem/5(PICCOLO_AP_MODE)
  Subsystem/3(Contact) -> Data Type Conversion/1, Gain/1
  Bus Creator/1 -> WOW_Bus_Out/1
  Data Type Conversion/1 -> Bus Creator/1  "ContactBool"
  Gain/1 -> Data Type Conversion1/1
  Data Type Conversion1/1 -> Bus Creator/2  "WoWPcnt"
  Data Type N/1 -> Delay3/1
  Data Type L/1 -> Delay1/1
  Re-Encoding L/1 -> Wheel to Cell Load MGL/1
  Software Saturation R/1 -> Re-Encoding R/1, Cell to Wheel Load MGR/1
  Signal Specification N/1 -> Software Saturation N/1
  Quantization L/1 -> Data Type L/1
  Quantization N/1 -> Data Type N/1
  Sum1/1 -> Quantization R/1
  Bus Element In1/1 -> Conversion - NG/1
  Sum/1 -> Quantization L/1
  Delay1/1 -> Signal Specification L/1
  Delay2/1 -> Signal Specification R/1
  DSC Noise N/1 -> Sum2/2
  Delay3/1 -> Signal Specification N/1
  Conversion - NG/1 -> Sum2/1
  Signal Specification L/1 -> Software Saturation L/1
  Cell to Wheel Load MGR/1 -> Subsystem/4(Sim.WOW_R_N)  "Sim.WOW_R_N"
  Quantization R/1 -> Data Type R/1
  Ground/1 -> Subsystem/3(RESET)
  Wheel to Cell Load MGR/1 -> Bus Creator1/3  "Sim.328_MGR_Cell_Telem_N"
  DSC Noise R/1 -> Sum1/2
  Software Saturation L/1 -> Re-Encoding L/1, Cell to Wheel Load MGL/1
  Data Type R/1 -> Delay2/1
  Cell to Wheel Load MGL/1 -> Subsystem/2(Sim.WOW_L_N)  "Sim.WOW_L_N"
  Sum2/1 -> Quantization N/1
  Re-Encoding R/1 -> Wheel to Cell Load MGR/1
  Bus Creator1/1 -> Terminator/1  "Sim.328_Integer_Loads"
  DSC Noise L/1 -> Sum/2
  Wheel to Cell Load MGL/1 -> Bus Creator1/2  "Sim.328_MGL_Cell_Telem_N"
  Cell to Wheel Load NG/1 -> Subsystem/1(Sim.WOW_NG_N)  "Sim.WOW_NG_N"
  Wheel to Cell Load NG/1 -> Bus Creator1/1  "Sim.328_NG_Cell_Telem_N"
  Software Saturation N/1 -> Re-Encoding N/1, Cell to Wheel Load NG/1
  Conversion - MGR/1 -> Sum1/1
  Signal Specification R/1 -> Software Saturation R/1
  Bus Element In5/1 -> Conversion - MGR/1
  Re-Encoding N/1 -> Wheel to Cell Load NG/1
  Bus Element In4/1 -> Conversion - MGL/1
  Conversion - MGL/1 -> Sum/1
